simulink model "vsi_02a_avg_pll"  (R2026a)
settings: Solver=FixedStepDiscrete  StopTime=Tstop  FixedStep=Ts
PostLoadFcn:
  | run(fullfile(fileparts(get_param('vsi_02a_avg_pll','FileName')), 'params_02a_avg_pll.m'));
InitFcn:
  | run(fullfile(fileparts(get_param('vsi_02a_avg_pll','FileName')), 'params_02a_avg_pll.m'));
values from neighbouring files (symbols this model uses):
  dw_max = 2*pi*5    (= 31.4159265359)    [params_02a_avg_pll.m]
  k_delay = 1.5    [params_02a_avg_pll.m]    (also in params_02c_switching.m = 2)
  Ki_pll = wn_pll^2    (= 15791.3670417)    [params_02a_avg_pll.m]
  Kp_pll = 2*zeta_pll*wn_pll    (= 177.688480487)    [params_02a_avg_pll.m]
  Tc = 1/fsw    [params_02a_avg_pll.m]
  Ts = Tc/20    [params_02a_avg_pll.m]    (also in params_02c_switching.m = Tc/200)
  vd_ref = sqrt(2)*real(E_pcc)    [params_02a_avg_pll.m]
  Vg_pk = sqrt(2)*Vg_ph    [params_02a_avg_pll.m]
  vq_ref = sqrt(2)*imag(E_pcc)    [params_02a_avg_pll.m]
undefined symbols (not defined in the file or in its folder): Lf, Lg, Rf, Rg, tau_pq, wg
libraries: ee_lib x4, nesl_utility x4, eeTransforms x2, fl_lib x2, eeGeneralControl x1, eeDiscretePi x1
settings Model: Creator=HAKAN SARI  LastModifiedBy=HAKAN SARI
settings SimscapeCC: SimscapeLogType=none

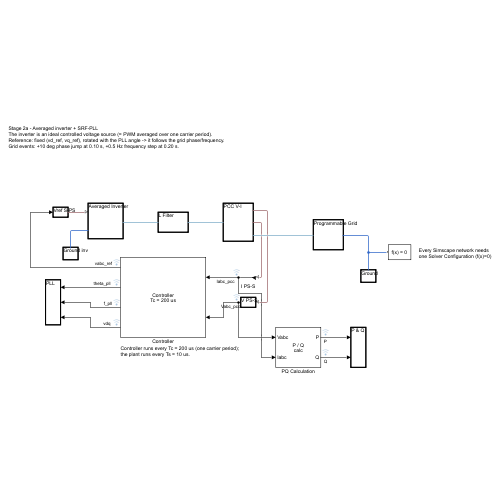
[thumbnail: Simulink's stored preview of the top-level diagram]
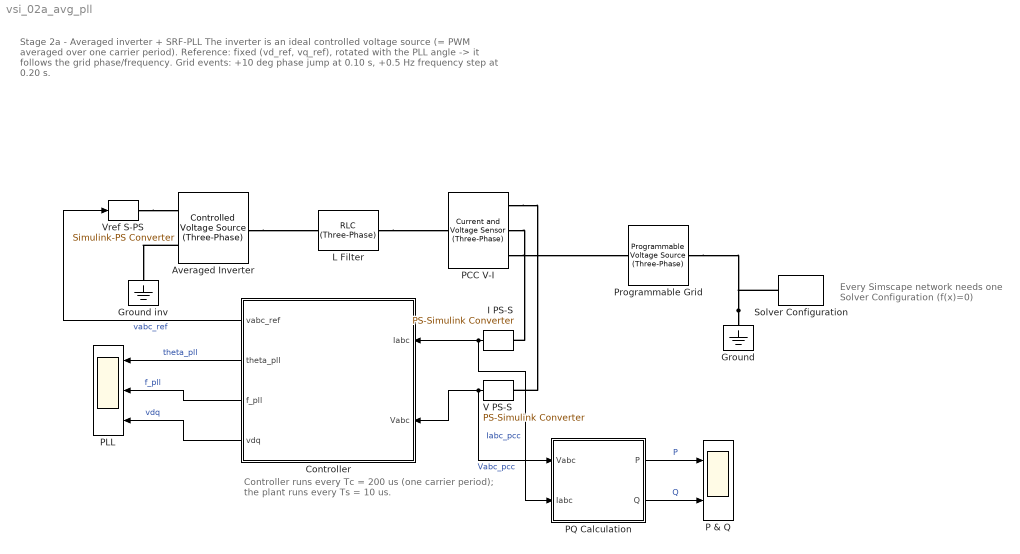
== system vsi_02a_avg_pll ==
  note: Stage 2a - Averaged inverter + SRF-PLL
      | The inverter is an ideal controlled voltage source (= PWM averaged over one carrier period).
      | Reference: fixed (vd_ref, vq_ref), rotated with the PLL angle -> it follows the grid phase/frequency.
      | Grid events: +10 deg phase jump at 0.10 s, +0.5 Hz frequency step at 0.20 s.
  note: Every Simscape network needs
      | one Solver Configuration (f(x)=0)
  note: Controller runs every Tc = 200 us (one carrier period);
      | the plant runs every Ts = 10 us.
  Averaged Inverter : ee_lib/Sources/Controlled Voltage Source (Three-Phase)  input_option=ee.enum.inputType.instantaneous  FRated=fg Hz
  Controller : Subsystem
      mask Display: disp('Controller\nTc = 200 us');
  Ground : fl_lib/Electrical/Electrical Elements/Electrical Reference
  Ground inv : fl_lib/Electrical/Electrical Elements/Electrical Reference
  I PS-S : nesl_utility/PS-Simulink Converter  PhysicalDomain=network_engine_domain  SubClassName=ps_output  LeftPortType=input  RightPortType=output  PseudoPeriodic=off  Frequencies=[]  VectorFormat=1-D array  Unit=inherit  AffineConversion=off
  L Filter : ee_lib/Passive/RLC Assemblies/RLC (Three-Phase)  port_option=ee.enum.threePhasePort.composite  component_structure=4  R=Rf Ohm  L=Lf H  C=1e-6 F  R_parasitic=0 Ohm  G_parasitic=0 1/Ohm  IL_specify=off  IL_priority=High  IL=[0, 0, 0] A  IL_nominal_specify=off  IL_nominal_value=1  IL_nominal_unit=A  VC_specify=off  VC_priority=High  VC=[0, 0, 0] V  VC_nominal_specify=off  VC_nominal_value=1  VC_nominal_unit=V
  P & Q : Scope  NumInputPorts=2
  PCC V-I : ee_lib/Sensors & Transducers/Current and Voltage Sensor (Three-Phase)  port_option=ee.enum.threePhasePort.composite  vMeasurementType=2  outputUnit=2  SRated=100e6 A*V  VRated=24e3 V  I_specify=off  I_priority=None  I=[0, 0, 0] A  I_nominal_specify=off  I_nominal_value=1  I_nominal_unit=A  V_specify=off  V_priority=None  V=[0, 0, 0] V  V_nominal_specify=off  V_nominal_value=1  V_nominal_unit=V
  PLL : Scope  NumInputPorts=3
  PQ Calculation : Subsystem
      mask Display: port_label('input',1,'Vabc');port_label('input',2,'Iabc');port_label('output',1,'P');port_label('output',2,'Q');disp('P / Q\ncalc');
  Programmable Grid : ee_lib/Sources/Programmable Voltage Source (Three-Phase)  magnitude_type=ee.enum.timechanging.constant  vline_rms=Vg_ll V  magn_ramp=1 V/s  magn_step=1 V  magn_modu_magn=1 V  magn_modu_freq=1 Hz  magn_t1=1 s  magn_t2=2 s  frequency_type=ee.enum.timechanging.step  freq=fg Hz  freq_ramp=1 Hz/s  freq_step=df_step Hz  freq_modu_magn=1 Hz  freq_modu_freq=1 Hz  freq_t1=t_freq s  freq_t2=inf s  phase_type=ee.enum.timechanging.step  shift=0 deg  phase_ramp=1 deg/s  phase_step=dphi_deg deg  phase_modu_magn=1 deg  phase_modu_freq=1 Hz  phase_t1=t_phase s  phase_t2=inf s  impedance_option=4  SShortCircuit=1e6 A*V  XR=15  R=Rg Ohm  L=Lg H  G_parasitic=1e-6 1/Ohm  harmonic_option=0  harmonic_orders=[5, 7, 11, 13]  harmonic_ratios=[.1, .1, .1, .1]  harmonic_shifts=[0, 0, 0, 0] deg  harmonic_sequences=[1, 1, 1, 1]  harmonic_t1=-inf s  harmonic_t2=inf s  I_specify=off  I_priority=None  I=[0, 0, 0] A  I_nominal_specify=off  I_nominal_value=1  I_nominal_unit=A  V_specify=off  V_priority=None  V=[0, 0, 0] V  V_nominal_specify=off  V_nominal_value=1  V_nominal_unit=V
  Solver Configuration : nesl_utility/Solver Configuration  PhysicalDomain=network_engine_domain  SubClassName=solver  LeftPortType=input  RightPortType=generic  Tones=[]  Harmonics=[]  SimulateNoise=off  Profile=off  UseLocalSampling=off  EnableSwitchedLinearOptims=on  FrequencyDomain=off  UseCCode=off  RelTol=0.001  AbsTol=0.001  MinStep=1e-09  ToWorkspace=off  RevertToSquareIcSolve=off  NumHomotopyIterations=100  PhasorMode=off  PhasorModeNumHarmonics=1  ConsistencySolver=NEWTON_XTOL_AFTER_FTOL  CanonicalOrdering=CANONICAL  OptimizeIntermediates=OPTIMIZED  IndexReductionMethod=DerivativeReplacement  DoDC=off  ResidualTolerance=1e-09  ConsistencyTolSource=GLOBAL  ConsistencyAbsTol=0.001  ConsistencyRelTol=0.001  ConsistencyTolFactor=0.001  UseLocalSolver=on  LocalSolverChoice=NE_BACKWARD_EULER_ADVANCER  ResolveIndetEquations=on  FunctionEvalNumThread=1  LocalSolverSampleTime=Ts  DoFixedCost=off  MaxNonlinIter=3  MaxModeIter=2  ComputeImpulses=off  ImpulseIterations=2  LinearAlgebra=auto  LinearAlgebraNumThread=0  EquationFormulation=NE_TIME_EF  DelaysMemoryBudget=1024  AutomaticFiltering=on  FilteringTimeConstant=0.001  PartitionStorageMethod=AS_NEEDED  PartitionMemoryBudget=1024  PartitionMethod=ROBUST  MultibodyUseLocalSolver=off  MultibodyLocalSolverChoice=ODE1  MultibodyLocalSolverSampleTime=0.001
  V PS-S : nesl_utility/PS-Simulink Converter  PhysicalDomain=network_engine_domain  SubClassName=ps_output  LeftPortType=input  RightPortType=output  PseudoPeriodic=off  Frequencies=[]  VectorFormat=1-D array  Unit=inherit  AffineConversion=off
  Vref S-PS : nesl_utility/Simulink-PS Converter  PhysicalDomain=network_engine_domain  SubClassName=ps_input  LeftPortType=input  RightPortType=output  PseudoPeriodic=off  Frequencies=[]  NoiseDistribution=none  NoiseParameters=[]  Unit=1  AffineConversion=off  FilteringAndDerivatives=zero  SimscapeFilterOrder=1  InputFilterTimeConstant=0.001  UdotUserProvided=0
  wires:
  I PS-S/1 -> Controller/1(Iabc), PQ Calculation/2(Iabc)  "Iabc_pcc"
  V PS-S/1 -> Controller/2(Vabc), PQ Calculation/1(Vabc)  "Vabc_pcc"
  Controller/1(vabc_ref) -> Vref S-PS/1  "vabc_ref"
  Controller/2(theta_pll) -> PLL/1  "theta_pll"
  Controller/3(f_pll) -> PLL/2  "f_pll"
  Controller/4(vdq) -> PLL/3  "vdq"
  PQ Calculation/1(P) -> P & Q/1  "P"
  PQ Calculation/2(Q) -> P & Q/2  "Q"
  connections:
  Averaged Inverter/LConn2 -- Ground inv/LConn1
  Vref S-PS/RConn1 -- Averaged Inverter/LConn1
  Averaged Inverter/RConn1 -- L Filter/LConn1
  L Filter/RConn1 -- PCC V-I/LConn1
  PCC V-I/RConn3 -- Programmable Grid/RConn1
  Ground/LConn1 -- Programmable Grid/LConn1 -- Solver Configuration/RConn1
  PCC V-I/RConn2 -- I PS-S/LConn1
  PCC V-I/RConn1 -- V PS-S/LConn1

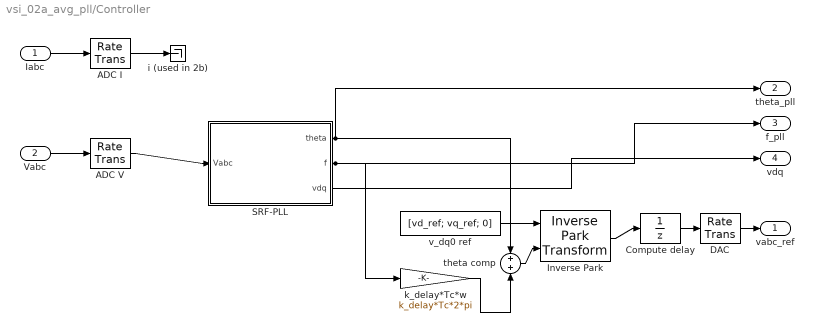
== system vsi_02a_avg_pll/Controller ==
  Iabc : Inport
  Vabc : Inport  Port=2
  ADC I : RateTransition  OutPortSampleTime=Tc
  ADC V : RateTransition  OutPortSampleTime=Tc
  Compute delay : UnitDelay  SampleTime=Tc
  DAC : RateTransition  Deterministic=off  OutPortSampleTime=Ts
  Inverse Park : eeTransforms/Inverse Park Transform  AxisAlignment=Q-axis  PowerInvariant=off
      settings: LibrarySourceBlock=|
      | ee_sl_lib/Mathematical
      | Transforms/Inverse
      | Park Transform
  SRF-PLL : Subsystem
      mask Display: disp('SRF-PLL');
  i (used in 2b) : Terminator
  k_delay*Tc*w : Gain  Gain=k_delay*Tc*2*pi
  theta comp : Sum
  v_dq0 ref : Constant  Value=[vd_ref; vq_ref; 0]
  vabc_ref : Outport
  theta_pll : Outport  Port=2
  f_pll : Outport  Port=3
  vdq : Outport  Port=4
  wires:
  Iabc/1 -> ADC I/1
  Vabc/1 -> ADC V/1
  ADC I/1 -> i (used in 2b)/1
  ADC V/1 -> SRF-PLL/1(Vabc)
  v_dq0 ref/1 -> Inverse Park/1
  SRF-PLL/2(f) -> k_delay*Tc*w/1, f_pll/1
  SRF-PLL/1(theta) -> theta comp/1, theta_pll/1
  k_delay*Tc*w/1 -> theta comp/2
  theta comp/1 -> Inverse Park/2
  Inverse Park/1 -> Compute delay/1
  Compute delay/1 -> DAC/1
  DAC/1 -> vabc_ref/1
  SRF-PLL/3(vdq) -> vdq/1

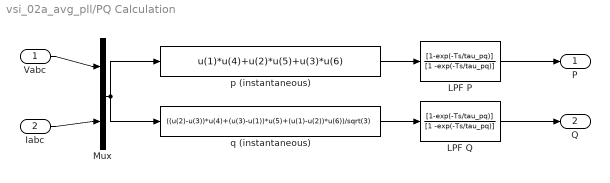
== system vsi_02a_avg_pll/PQ Calculation ==
  Vabc : Inport
  Iabc : Inport  Port=2
  LPF P : DiscreteTransferFcn  Numerator=[1-exp(-Ts/tau_pq)]  Denominator=[1 -exp(-Ts/tau_pq)]  SampleTime=Ts
  LPF Q : DiscreteTransferFcn  Numerator=[1-exp(-Ts/tau_pq)]  Denominator=[1 -exp(-Ts/tau_pq)]  SampleTime=Ts
  Mux : Mux  Inputs=2
  p (instantaneous) : Fcn  Expr=u(1)*u(4)+u(2)*u(5)+u(3)*u(6)
  q (instantaneous) : Fcn  Expr=((u(2)-u(3))*u(4)+(u(3)-u(1))*u(5)+(u(1)-u(2))*u(6))/sqrt(3)
  P : Outport
  Q : Outport  Port=2
  wires:
  Vabc/1 -> Mux/1
  Iabc/1 -> Mux/2
  Mux/1 -> p (instantaneous)/1, q (instantaneous)/1
  p (instantaneous)/1 -> LPF P/1
  q (instantaneous)/1 -> LPF Q/1
  LPF P/1 -> P/1
  LPF Q/1 -> Q/1

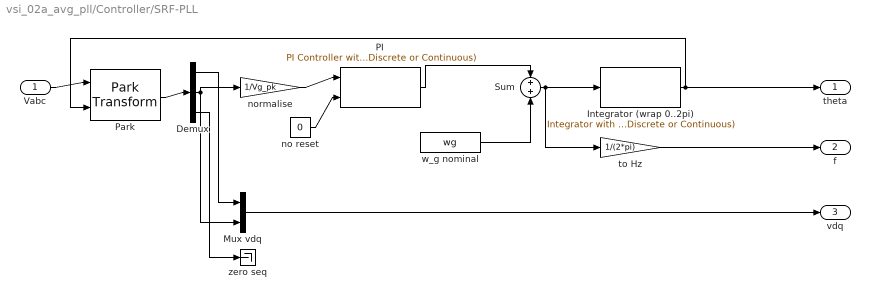
== system vsi_02a_avg_pll/Controller/SRF-PLL ==
  Vabc : Inport
  Demux : Demux  Outputs=3
  Integrator (wrap 0..2pi) : eeGeneralControl/Integrator with Wrapped State (Discrete or Continuous)  LabelModeActiveChoice=Discrete  WrappedStateUpperValue=2*pi  WrappedStateLowerValue=0  x0=0  Ts=Tc
      settings: LibrarySourceBlock=|
      | ee_sl_lib/General Control/Integrator with
      | Wrapped State
      | (Discrete or Continuous)
  Mux vdq : Mux  Inputs=2
  PI : eeDiscretePi/PI Controller with Integral Anti-Windup (Discrete or Continuous)  Kp=Kp_pll  Ki=Ki_pll  x0=0  B=dw_max  A=-dw_max  Ts=Tc
      settings: LibrarySourceBlock=|
      | ee_sl_lib/General Control/PI Controller with
      | Integral Anti-Windup
      | (Discrete or Continuous)
  Park : eeTransforms/Park Transform  AxisAlignment=Q-axis  PowerInvariant=off
      settings: LibrarySourceBlock=|
      | ee_sl_lib/Mathematical
      | Transforms/Park Transform
  Sum : Sum
  no reset : Constant  Value=0  SampleTime=Tc
  normalise : Gain  Gain=1/Vg_pk
  to Hz : Gain  Gain=1/(2*pi)
  w_g nominal : Constant  Value=wg  SampleTime=Tc
  zero seq : Terminator
  theta : Outport
  f : Outport  Port=2
  vdq : Outport  Port=3
  wires:
  Vabc/1 -> Park/1
  Park/1 -> Demux/1
  Demux/2 -> normalise/1, Mux vdq/2
  normalise/1 -> PI/1
  no reset/1 -> PI/2
  PI/1 -> Sum/1
  w_g nominal/1 -> Sum/2
  Sum/1 -> Integrator (wrap 0..2pi)/1, to Hz/1
  Integrator (wrap 0..2pi)/1 -> theta/1, Park/2
  to Hz/1 -> f/1
  Demux/1 -> Mux vdq/1
  Demux/3 -> zero seq/1
  Mux vdq/1 -> vdq/1
